simulink model "VisionSystem_Behavior"  (R2025b)
settings: Solver=VariableStepAuto  StartTime=0.0  StopTime=10.0  RelTol=1e-3
settings Model: Creator=prati  LastModifiedBy=prati

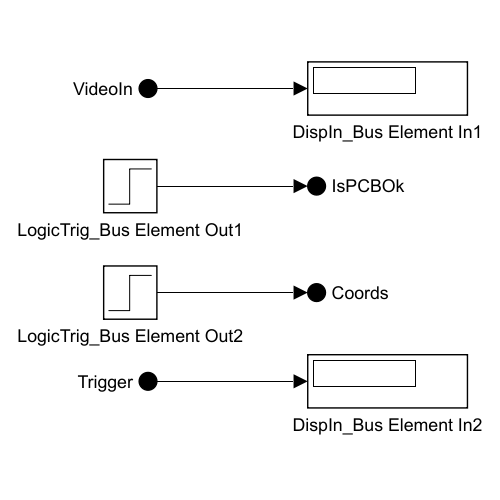
[thumbnail: Simulink's stored preview of the top-level diagram]
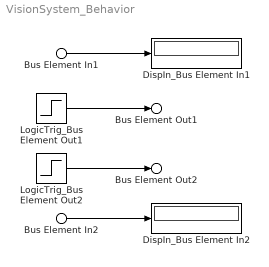
== system VisionSystem_Behavior ==
  Bus Element In1 : Inport  PortName=VideoIn
  Bus Element In2 : Inport  Port=2  PortName=Trigger
  DispIn_Bus Element In1 : Display
  DispIn_Bus Element In2 : Display
  LogicTrig_Bus Element Out1 : Step  Time=0  SampleTime=0
  LogicTrig_Bus Element Out2 : Step  Time=0  SampleTime=0
  Bus Element Out1 : Outport  PortName=IsPCBOk
  Bus Element Out2 : Outport  Port=2  PortName=Coords
  wires:
  Bus Element In1/1 -> DispIn_Bus Element In1/1
  Bus Element In2/1 -> DispIn_Bus Element In2/1
  LogicTrig_Bus Element Out1/1 -> Bus Element Out1/1
  LogicTrig_Bus Element Out2/1 -> Bus Element Out2/1
